simulink model "chbtask"  (R2024b)
settings: Solver=FixedStepDiscrete  StartTime=0.0  StopTime=0.2  FixedStep=5e-5  RelTol=1e-3
values from neighbouring files (symbols this model uses):
  CHB_MODE : value not decoded    [CHB_Data.sldd]
  INV120_CUURENTLOOP_KP = 2.0    [CHB_Data.sldd]
  INV120_CUURENTLOOP_KR = 5.0    [CHB_Data.sldd]
  INV120_VOLTAGELOOP_KI = 0.005    [CHB_Data.sldd]
  INV120_VOLTAGELOOP_KP = 0.5    [CHB_Data.sldd]
  INV240_VOLTAGELOOP_KI = 0.005    [CHB_Data.sldd]
  INV240_VOLTAGELOOP_KP = 0.5    [CHB_Data.sldd]
  PFC120_CUURENTLOOP_KP = 30.0    [CHB_Data.sldd]
  PFC120_CUURENTLOOP_KR = 8.0    [CHB_Data.sldd]
  PFC120_POWERLOOP_KI = 0.0001    [CHB_Data.sldd]
  PFC120_POWERLOOP_KP = 0.005    [CHB_Data.sldd]
  PFC240_CUURENTLOOP_KP = 5.0    [CHB_Data.sldd]
  PFC240_CUURENTLOOP_KR = 10.0    [CHB_Data.sldd]
  PFC240_POWERLOOP_KI = 0.0001    [CHB_Data.sldd]
  PFC240_POWERLOOP_KP = 0.005    [CHB_Data.sldd]
undefined symbols (not defined in the file or in its folder): Ii_rms, Io_rms, Io_rms_a, Io_rms_b, Vi_freq, Vi_rms, Vo_freq, Vo_freq_a, Vo_freq_b, Vo_rms, Vo_rms_a, Vo_rms_b
(part 2 of 3)

== system chbtask/Algorithm_Ctrl/MainCtrl/inv240_func/inv240_en ==
  note: 抗积分饱和
  note: 峰值限流保护是什么？？
  Bus Element In1 : Inport  PortName=Algorithm  Element=Vo_rms
  Enable : EnablePort
  Chart : Stateflow chart  TreatAsAtomicUnit=on
  Constant : Constant  Value=240  OutDataTypeStr=single
  Constant1 : Constant  Value=INV240_VOLTAGELOOP_KP  OutDataTypeStr=single
  Constant2 : Constant  Value=INV240_VOLTAGELOOP_KI  OutDataTypeStr=single
  Constant3 : Constant  Value=[360 100]  OutDataTypeStr=single
  Delay : Delay  DelayLength=1  InputProcessing=Columns as channels (frame based)
  Function Caller : FunctionCaller  FunctionPrototype=PI_out = Func.PI_Ctrl(error,err_sum,Kp,Ki,out_limit)  InputArgumentSpecifications=<Enter example>  OutputArgumentSpecifications=<Enter example>
  Mux : Mux  Inputs=2
  Saturation : Saturate  UpperLimit=360/INV240_VOLTAGELOOP_KI  LowerLimit=100/INV240_VOLTAGELOOP_KI
  Sum : Sum  Inputs=+-|
  Sum1 : Sum  Inputs=++|
  duty : Outport  OutDataTypeStr=single  PortDimensions=[1 2]
  wires:
  Constant/1 -> Sum/1
  Sum/1 -> Sum1/1, Function Caller/1
  Constant1/1 -> Function Caller/3
  Constant2/1 -> Function Caller/4
  Delay/1 -> Sum1/2
  Sum1/1 -> Saturation/1
  Constant3/1 -> Function Caller/5
  Function Caller/1 -> Chart/1(Pi_inv_out)
  Bus Element In1/1 -> Sum/2
  Mux/1 -> duty/1
  Chart/1(out) -> Mux/1, Mux/2
  Saturation/1 -> Delay/1, Function Caller/2

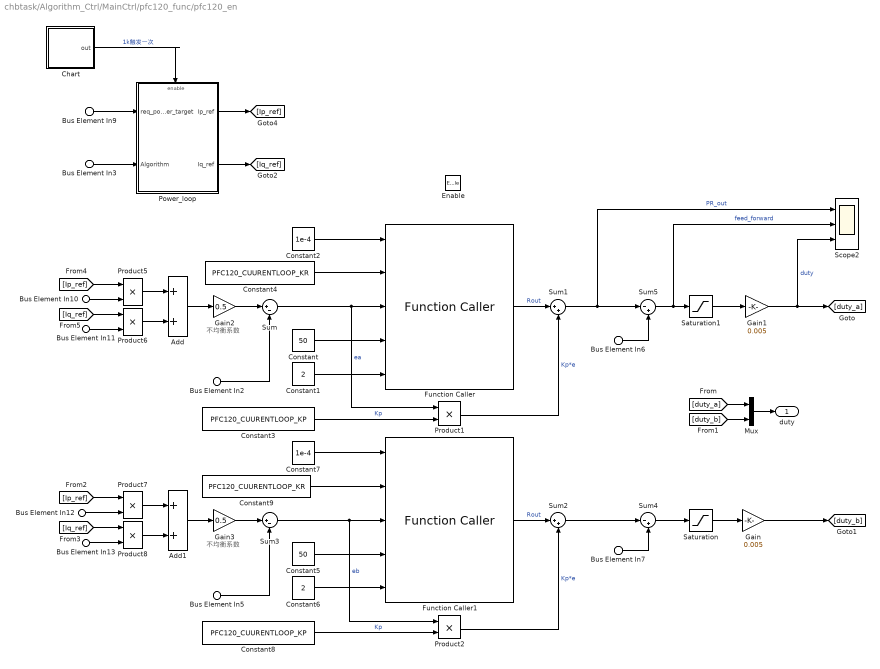
== system chbtask/Algorithm_Ctrl/MainCtrl/pfc120_func/pfc120_en ==
  note: 不均衡系数
  note: 不均衡系数
  Bus Element In10 : Inport  PortName=PLL  Element=cosin
  Bus Element In12 : Inport  PortName=PLL  Element=cosin
  Bus Element In11 : Inport  PortName=PLL  Element=sine
  Bus Element In13 : Inport  PortName=PLL  Element=sine
  Bus Element In2 : Inport  Port=2  PortName=Sampling  Element=AC_in_A.Igrid
  Bus Element In5 : Inport  Port=2  PortName=Sampling  Element=AC_in_B.Igrid
  Bus Element In6 : Inport  Port=2  PortName=Sampling  Element=AC_in.Vgrid
  Bus Element In7 : Inport  Port=2  PortName=Sampling  Element=AC_in.Vgrid
  Bus Element In9 : Inport  Port=2  PortName=Sampling  Element=AC_in.Power
  Bus Element In3 : Inport  Port=3  PortName=Algorithm
  Enable : EnablePort
  Add : Sum  OutDataTypeStr=single  AccumDataTypeStr=single
  Add1 : Sum  OutDataTypeStr=single  AccumDataTypeStr=single
  Chart : Stateflow chart  TreatAsAtomicUnit=on
  Constant : Constant  Value=50  OutDataTypeStr=single
  Constant1 : Constant  Value=2  OutDataTypeStr=single
  Constant2 : Constant  Value=1e-4  OutDataTypeStr=single
  Constant3 : Constant  Value=PFC120_CUURENTLOOP_KP  OutDataTypeStr=single
  Constant4 : Constant  Value=PFC120_CUURENTLOOP_KR  OutDataTypeStr=single
  Constant5 : Constant  Value=50  OutDataTypeStr=single
  Constant6 : Constant  Value=2  OutDataTypeStr=single
  Constant7 : Constant  Value=1e-4  OutDataTypeStr=single
  Constant8 : Constant  Value=PFC120_CUURENTLOOP_KP  OutDataTypeStr=single
  Constant9 : Constant  Value=PFC120_CUURENTLOOP_KR  OutDataTypeStr=single
  Function Caller : FunctionCaller  FunctionPrototype=R_out = Func.R_Ctrl(Ts,Kr,uk,freq0,freqc)  InputArgumentSpecifications=<Enter example>  OutputArgumentSpecifications=<Enter example>
  Function Caller1 : FunctionCaller  FunctionPrototype=R_out = Func.R_Ctrl(Ts,Kr,uk,freq0,freqc)  InputArgumentSpecifications=<Enter example>  OutputArgumentSpecifications=<Enter example>
  Gain : Gain  Gain=0.005  OutDataTypeStr=single
  Gain1 : Gain  Gain=0.005  OutDataTypeStr=single
  Gain2 : Gain  Gain=0.5  OutDataTypeStr=single
  Gain3 : Gain  Gain=0.5  OutDataTypeStr=single
  Mux : Mux  Inputs=2
  Power_loop : Subsystem
  Product1 : Product
  Product2 : Product
  Product{5..8} (4 alike) : Product  OutDataTypeStr=single
  Saturation : Saturate  UpperLimit=200  LowerLimit=-200  OutDataTypeStr=single
  Saturation1 : Saturate  UpperLimit=200  LowerLimit=-200  OutDataTypeStr=single
  Scope2 : Scope  NumInputPorts=3
  Sum : Sum  Inputs=|+-  OutDataTypeStr=single  AccumDataTypeStr=single
  Sum1 : Sum  Inputs=|++  OutDataTypeStr=single  AccumDataTypeStr=single
  Sum2 : Sum  Inputs=|++  OutDataTypeStr=single  AccumDataTypeStr=single
  Sum3 : Sum  Inputs=|+-
  Sum4 : Sum  Inputs=|-+  OutDataTypeStr=single  AccumDataTypeStr=single
  Sum5 : Sum  Inputs=|-+  OutDataTypeStr=single  AccumDataTypeStr=single
  duty : Outport  OutDataTypeStr=single  PortDimensions=[1 2]
  wires:
  Constant3/1 -> Product1/2  "Kp"
  Product1/1 -> Sum1/2  "Kp*e"
  Constant2/1 -> Function Caller/1
  Constant4/1 -> Function Caller/2
  Function Caller/1 -> Sum1/1  "Rout"
  Constant/1 -> Function Caller/4
  Constant1/1 -> Function Caller/5
  Constant6/1 -> Function Caller1/5
  Constant5/1 -> Function Caller1/4
  Function Caller1/1 -> Sum2/1  "Rout"
  Constant9/1 -> Function Caller1/2
  Constant7/1 -> Function Caller1/1
  Product2/1 -> Sum2/2  "Kp*e"
  Constant8/1 -> Product2/2  "Kp"
  Sum/1 -> Product1/1, Function Caller/3  "ea"
  Bus Element In2/1 -> Sum/2
  Sum3/1 -> Product2/1, Function Caller1/3  "eb"
  Bus Element In5/1 -> Sum3/2
  Mux/1 -> duty/1
  [duty_a] -> Mux/1
  [duty_b] -> Mux/2
  Sum2/1 -> Sum4/1
  Bus Element In7/1 -> Sum4/2
  Sum1/1 -> Scope2/1, Sum5/1  "PR_out"
  Bus Element In6/1 -> Sum5/2
  Saturation/1 -> Gain/1
  Sum4/1 -> Saturation/1
  Saturation1/1 -> Gain1/1
  Gain1/1 -> [duty_a], Scope2/3  "duty"
  Gain/1 -> [duty_b]
  Sum5/1 -> Scope2/2, Saturation1/1  "feed_forward"
  Chart/1(out) -> Power_loop/Enable  "1k触发一次"
  Bus Element In3/1 -> Power_loop/2(Algorithm)
  Bus Element In9/1 -> Power_loop/1(req_power_target)
  Bus Element In11/1 -> Product6/2
  Product6/1 -> Add/2
  Product5/1 -> Add/1
  [Iq_ref] -> Product6/1
  [Ip_ref] -> Product5/1
  Bus Element In10/1 -> Product5/2
  Power_loop/2(Iq_ref) -> [Iq_ref]
  Power_loop/1(Ip_ref) -> [Ip_ref]
  Add/1 -> Gain2/1
  Gain2/1 -> Sum/1
  Add1/1 -> Gain3/1
  Bus Element In12/1 -> Product7/2
  [Ip_ref] -> Product7/1
  [Iq_ref] -> Product8/1
  Product7/1 -> Add1/1
  Product8/1 -> Add1/2
  Bus Element In13/1 -> Product8/2
  Gain3/1 -> Sum3/1

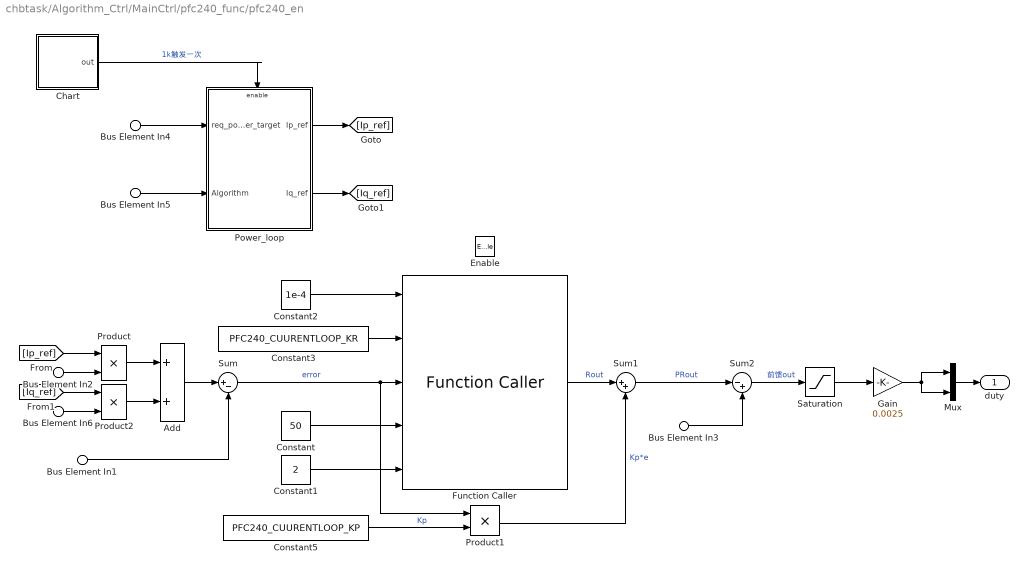
== system chbtask/Algorithm_Ctrl/MainCtrl/pfc240_func/pfc240_en ==
  Bus Element In2 : Inport  PortName=PLL  Element=cosin
  Bus Element In6 : Inport  PortName=PLL  Element=sine
  Bus Element In1 : Inport  Port=2  PortName=Sampling  Element=AC_in.Igrid
  Bus Element In3 : Inport  Port=2  PortName=Sampling  Element=AC_in.Vgrid
  Bus Element In4 : Inport  Port=2  PortName=Sampling  Element=AC_in.Power
  Bus Element In5 : Inport  Port=3  PortName=Algorithm
  Enable : EnablePort
  Add : Sum
  Chart : Stateflow chart  TreatAsAtomicUnit=on
  Constant : Constant  Value=50  OutDataTypeStr=single
  Constant1 : Constant  Value=2  OutDataTypeStr=single
  Constant2 : Constant  Value=1e-4  OutDataTypeStr=single
  Constant3 : Constant  Value=PFC240_CUURENTLOOP_KR  OutDataTypeStr=single
  Constant5 : Constant  Value=PFC240_CUURENTLOOP_KP  OutDataTypeStr=single
  Function Caller : FunctionCaller  FunctionPrototype=R_out = Func.R_Ctrl(Ts,Kr,uk,freq0,freqc)  InputArgumentSpecifications=<Enter example>  OutputArgumentSpecifications=<Enter example>
  Gain : Gain  Gain=0.0025  OutDataTypeStr=single
  Mux : Mux  Inputs=2
  Power_loop : Subsystem
  Product : Product  OutDataTypeStr=single
  Product1 : Product
  Product2 : Product  OutDataTypeStr=single
  Saturation : Saturate  UpperLimit=400  LowerLimit=-400  OutDataTypeStr=single
  Sum : Sum  Inputs=|+-  OutDataTypeStr=single  AccumDataTypeStr=single
  Sum1 : Sum  Inputs=|++  OutDataTypeStr=single  AccumDataTypeStr=single
  Sum2 : Sum  Inputs=|-+
  duty : Outport  OutDataTypeStr=single  PortDimensions=[1 2]
  wires:
  Constant1/1 -> Function Caller/5
  Constant/1 -> Function Caller/4
  Constant2/1 -> Function Caller/1
  Constant3/1 -> Function Caller/2
  Sum/1 -> Product1/1, Function Caller/3  "error"
  Bus Element In2/1 -> Product/2
  Constant5/1 -> Product1/2  "Kp"
  Function Caller/1 -> Sum1/1  "Rout"
  Product1/1 -> Sum1/2  "Kp*e"
  Saturation/1 -> Gain/1
  Sum1/1 -> Sum2/1  "PRout"
  Sum2/1 -> Saturation/1  "前馈out"
  Chart/1(out) -> Power_loop/Enable  "1k触发一次"
  Bus Element In1/1 -> Sum/2
  Bus Element In3/1 -> Sum2/2
  Bus Element In4/1 -> Power_loop/1(req_power_target)
  Bus Element In5/1 -> Power_loop/2(Algorithm)
  Power_loop/1(Ip_ref) -> [Ip_ref]
  [Ip_ref] -> Product/1
  Power_loop/2(Iq_ref) -> [Iq_ref]
  Bus Element In6/1 -> Product2/2
  Product2/1 -> Add/2
  Product/1 -> Add/1
  Add/1 -> Sum/1
  [Iq_ref] -> Product2/1
  Mux/1 -> duty/1
  Gain/1 -> Mux/2, Mux/1

== system chbtask/Algorithm_Ctrl/MainCtrl/inv120_func/inv120_en/Power_loop ==
  Vo_rms : Inport  OutDataTypeStr=single
  Enable : EnablePort
  Constant : Constant  Value=120  OutDataTypeStr=single
  Constant1 : Constant  Value=INV120_VOLTAGELOOP_KP  OutDataTypeStr=single
  Constant2 : Constant  Value=INV120_VOLTAGELOOP_KI  OutDataTypeStr=single
  Constant3 : Constant  Value=[30 0]  OutDataTypeStr=single
  Delay : Delay  DelayLength=1  InputProcessing=Columns as channels (frame based)
  Function Caller : FunctionCaller  FunctionPrototype=PI_out = Func.PI_Ctrl(error,err_sum,Kp,Ki,out_limit)  InputArgumentSpecifications=<Enter example>  OutputArgumentSpecifications=<Enter example>
  Scope : Scope
  Sum : Sum  Inputs=+-|
  Sum1 : Sum  Inputs=++|
  itotal_rms : Outport
  wires:
  Vo_rms/1 -> Sum/2
  Delay/1 -> Sum1/2
  Constant/1 -> Sum/1
  Constant3/1 -> Function Caller/5
  Sum1/1 -> Delay/1, Function Caller/2
  Sum/1 -> Sum1/1, Function Caller/1
  Function Caller/1 -> itotal_rms/1, Scope/1
  Constant2/1 -> Function Caller/4
  Constant1/1 -> Function Caller/3

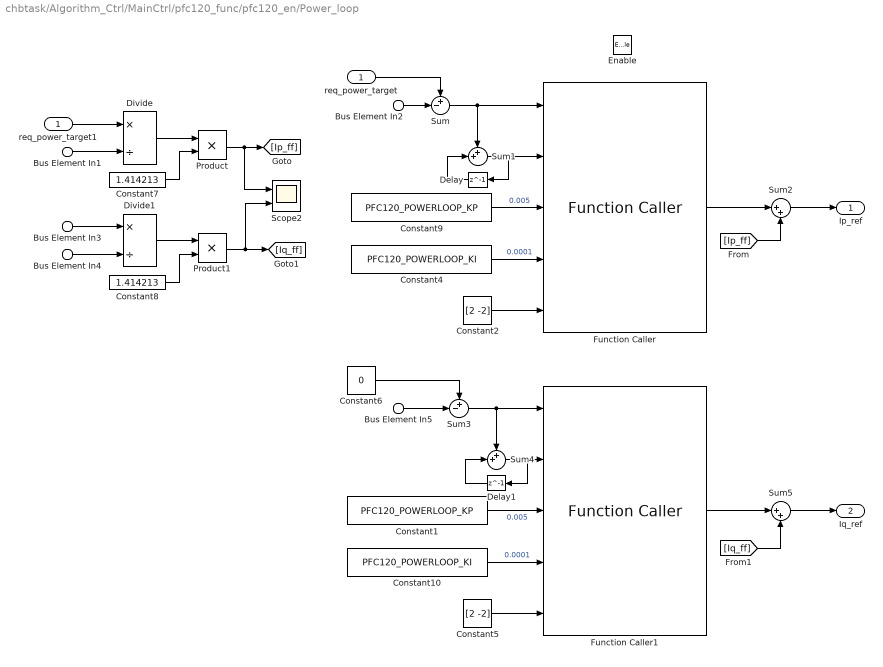
== system chbtask/Algorithm_Ctrl/MainCtrl/pfc120_func/pfc120_en/Power_loop ==
  req_power_target : Inport
  Bus Element In2 : Inport  Port=2  PortName=Algorithm  Element=pfc.P
  Bus Element In3 : Inport  Port=2  PortName=Algorithm  Element=pfc.Q
  Bus Element In5 : Inport  Port=2  PortName=Algorithm  Element=pfc.Q
  Bus Element In1 : Inport  Port=2  PortName=Algorithm  Element=Vi_rms
  Bus Element In4 : Inport  Port=2  PortName=Algorithm  Element=Vi_rms
  Enable : EnablePort
  Constant1 : Constant  Value=PFC120_POWERLOOP_KP  OutDataTypeStr=single
  Constant10 : Constant  Value=PFC120_POWERLOOP_KI  OutDataTypeStr=single
  Constant2 : Constant  Value=[2 -2]  OutDataTypeStr=single
  Constant4 : Constant  Value=PFC120_POWERLOOP_KI  OutDataTypeStr=single
  Constant5 : Constant  Value=[2 -2]  OutDataTypeStr=single
  Constant6 : Constant  Value=0  OutDataTypeStr=single
  Constant7 : Constant  Value=1.414213  OutDataTypeStr=single
  Constant8 : Constant  Value=1.414213  OutDataTypeStr=single
  Constant9 : Constant  Value=PFC120_POWERLOOP_KP  OutDataTypeStr=single
  Delay : Delay  DelayLength=1  InputProcessing=Columns as channels (frame based)
  Delay1 : Delay  DelayLength=1  InputProcessing=Columns as channels (frame based)
  Divide : Product  Inputs=*/  OutDataTypeStr=single
  Divide1 : Product  Inputs=*/  OutDataTypeStr=single
  Function Caller : FunctionCaller  FunctionPrototype=PI_out = Func.PI_Ctrl(error,err_sum,Kp,Ki,out_limit)  InputArgumentSpecifications=<Enter example>  OutputArgumentSpecifications=<Enter example>
  Function Caller1 : FunctionCaller  FunctionPrototype=PI_out = Func.PI_Ctrl(error,err_sum,Kp,Ki,out_limit)  InputArgumentSpecifications=<Enter example>  OutputArgumentSpecifications=<Enter example>
  Product : Product  OutDataTypeStr=single
  Product1 : Product  OutDataTypeStr=single
  Scope2 : Scope  NumInputPorts=2
  Sum : Sum  Inputs=+-|  OutDataTypeStr=single
  Sum1 : Sum  Inputs=++|  OutDataTypeStr=single
  Sum2 : Sum  Inputs=|++
  Sum3 : Sum  Inputs=+-|  OutDataTypeStr=single
  Sum4 : Sum  Inputs=++|  OutDataTypeStr=single
  Sum5 : Sum  Inputs=|++
  req_power_target1 : InportShadow
  Ip_ref : Outport
  Iq_ref : Outport  Port=2
  wires:
  Bus Element In2/1 -> Sum/2
  req_power_target/1 -> Sum/1
  Sum/1 -> Sum1/1, Function Caller/1
  Sum1/1 -> Delay/1, Function Caller/2
  Delay/1 -> Sum1/2
  Constant9/1 -> Function Caller/3  "0.005"
  Constant4/1 -> Function Caller/4  "0.0001"
  Constant2/1 -> Function Caller/5
  req_power_target1/1 -> Divide/1
  Bus Element In1/1 -> Divide/2
  Constant5/1 -> Function Caller1/5
  Delay1/1 -> Sum4/2
  Sum4/1 -> Function Caller1/2, Delay1/1
  Sum3/1 -> Function Caller1/1, Sum4/1
  Constant6/1 -> Sum3/1
  Bus Element In5/1 -> Sum3/2
  Bus Element In3/1 -> Divide1/1
  Bus Element In4/1 -> Divide1/2
  Function Caller1/1 -> Sum5/1
  [Iq_ff] -> Sum5/2
  Sum2/1 -> Ip_ref/1
  Function Caller/1 -> Sum2/1
  [Ip_ff] -> Sum2/2
  Divide/1 -> Product/1
  Constant7/1 -> Product/2
  Product/1 -> Scope2/1, [Ip_ff]
  Constant8/1 -> Product1/2
  Divide1/1 -> Product1/1
  Product1/1 -> Scope2/2, [Iq_ff]
  Sum5/1 -> Iq_ref/1
  Constant10/1 -> Function Caller1/4  "0.0001"
  Constant1/1 -> Function Caller1/3  "0.005"

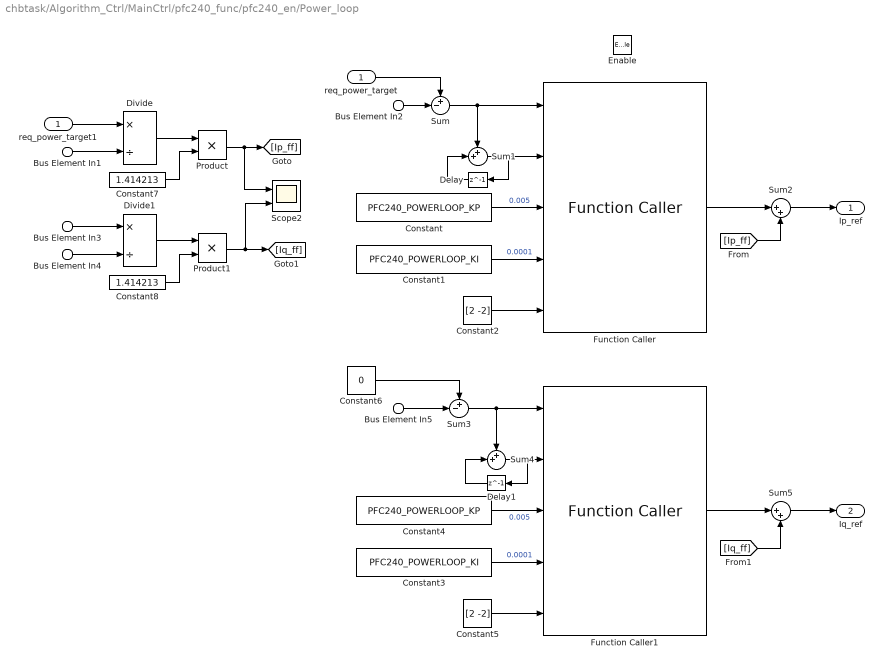
== system chbtask/Algorithm_Ctrl/MainCtrl/pfc240_func/pfc240_en/Power_loop ==
  req_power_target : Inport
  Bus Element In2 : Inport  Port=2  PortName=Algorithm  Element=pfc.P
  Bus Element In3 : Inport  Port=2  PortName=Algorithm  Element=pfc.Q
  Bus Element In5 : Inport  Port=2  PortName=Algorithm  Element=pfc.Q
  Bus Element In1 : Inport  Port=2  PortName=Algorithm  Element=Vi_rms
  Bus Element In4 : Inport  Port=2  PortName=Algorithm  Element=Vi_rms
  Enable : EnablePort
  Constant : Constant  Value=PFC240_POWERLOOP_KP  OutDataTypeStr=single
  Constant1 : Constant  Value=PFC240_POWERLOOP_KI  OutDataTypeStr=single
  Constant2 : Constant  Value=[2 -2]  OutDataTypeStr=single
  Constant3 : Constant  Value=PFC240_POWERLOOP_KI  OutDataTypeStr=single
  Constant4 : Constant  Value=PFC240_POWERLOOP_KP  OutDataTypeStr=single
  Constant5 : Constant  Value=[2 -2]  OutDataTypeStr=single
  Constant6 : Constant  Value=0  OutDataTypeStr=single
  Constant7 : Constant  Value=1.414213  OutDataTypeStr=single
  Constant8 : Constant  Value=1.414213  OutDataTypeStr=single
  Delay : Delay  DelayLength=1  InputProcessing=Columns as channels (frame based)
  Delay1 : Delay  DelayLength=1  InputProcessing=Columns as channels (frame based)
  Divide : Product  Inputs=*/  OutDataTypeStr=single
  Divide1 : Product  Inputs=*/  OutDataTypeStr=single
  Function Caller : FunctionCaller  FunctionPrototype=PI_out = Func.PI_Ctrl(error,err_sum,Kp,Ki,out_limit)  InputArgumentSpecifications=<Enter example>  OutputArgumentSpecifications=<Enter example>
  Function Caller1 : FunctionCaller  FunctionPrototype=PI_out = Func.PI_Ctrl(error,err_sum,Kp,Ki,out_limit)  InputArgumentSpecifications=<Enter example>  OutputArgumentSpecifications=<Enter example>
  Product : Product  OutDataTypeStr=single
  Product1 : Product  OutDataTypeStr=single
  Scope2 : Scope  NumInputPorts=2
  Sum : Sum  Inputs=+-|  OutDataTypeStr=single
  Sum1 : Sum  Inputs=++|  OutDataTypeStr=single
  Sum2 : Sum  Inputs=|++
  Sum3 : Sum  Inputs=+-|  OutDataTypeStr=single
  Sum4 : Sum  Inputs=++|  OutDataTypeStr=single
  Sum5 : Sum  Inputs=|++
  req_power_target1 : InportShadow
  Ip_ref : Outport
  Iq_ref : Outport  Port=2
  wires:
  Bus Element In2/1 -> Sum/2
  req_power_target/1 -> Sum/1
  Sum/1 -> Sum1/1, Function Caller/1
  Sum1/1 -> Delay/1, Function Caller/2
  Delay/1 -> Sum1/2
  Constant/1 -> Function Caller/3  "0.005"
  Constant1/1 -> Function Caller/4  "0.0001"
  Constant2/1 -> Function Caller/5
  req_power_target1/1 -> Divide/1
  Bus Element In1/1 -> Divide/2
  Constant5/1 -> Function Caller1/5
  Delay1/1 -> Sum4/2
  Sum4/1 -> Function Caller1/2, Delay1/1
  Sum3/1 -> Function Caller1/1, Sum4/1
  Constant6/1 -> Sum3/1
  Bus Element In5/1 -> Sum3/2
  Bus Element In3/1 -> Divide1/1
  Bus Element In4/1 -> Divide1/2
  Function Caller1/1 -> Sum5/1
  [Iq_ff] -> Sum5/2
  Sum2/1 -> Ip_ref/1
  Function Caller/1 -> Sum2/1
  [Ip_ff] -> Sum2/2
  Divide/1 -> Product/1
  Constant7/1 -> Product/2
  Product/1 -> Scope2/1, [Ip_ff]
  Constant8/1 -> Product1/2
  Divide1/1 -> Product1/1
  Product1/1 -> Scope2/2, [Iq_ff]
  Sum5/1 -> Iq_ref/1
  Constant3/1 -> Function Caller1/4  "0.0001"
  Constant4/1 -> Function Caller1/3  "0.005"

== stateflow chart chbtask/Algorithm_Ctrl/Data treating/SOGI/SOGI_Core ==
  state Run
    du:
    omega = 2*pi*single(50);
    T = single(1e-4);
    k = single(sqrt(2));
    e = vac - alpha_1 - k*beta_1;
    v_alpha = alpha_1 + T*omega*e;
    v_beta  = beta_1 + T*omega*v_alpha;
    alpha_1 = v_alpha;
    beta_1  = v_beta;
  (default) -> Run
  data: alpha_1 local single =0; beta_1 local single =0; omega local single =single(2*pi*50); T local single =single(1e-4); k local single =single(sqrt(2)); e local single; vac input single; v_alpha output single; v_beta output single

== stateflow chart chbtask/Algorithm_Ctrl/MainCtrl/pfc240_func/pfc240_en/Chart ==
  (default) -> (junction 8)
  (junction 8) -> (junction 6) [order 1] : [cnt>=9]
  (junction 8) -> (junction 10) [order 2] : {
      | out=0;
      | cnt = cnt + 1;
      | }
  (junction 6) -> (junction 11) : {
      | out=1;
      | cnt = 0;
      | }
  (junction 10) -> (junction 11)
  (junction 11) -> (junction 23)
  data: cnt local uint16 =0; out output uint16

== stateflow chart chbtask/Algorithm_Ctrl/MainCtrl/inv240_func/inv240_en/Chart ==
  (default) -> (junction 3) : {
      | pi_out_value = single(0.0025)*Pi_inv_out;
      | cnt = mod(cnt + 1, 200);
      | %PWM1 = sin_tab(mod(cnt + 0, 400) + 1);
      | out = pi_out_value*sin_wave(mod(cnt + 0, 200) + 1);
      | }
  data: sin_wave local single =[
0.000000000, 0.031410759, 0.062790520, 0.094108313, 0.125333234, 0.156434465, 0.187381315, 0.218143241, 0.248689887, 0.278991106, 0.309016994, 0.338737920, 0.368124553, 0.397147891, 0.425779292, 0.453990500, 0.481753674, 0.509041416, 0.535826795, 0.562083325, 0.587785252, 0.612907054, 0.637423990, 0.661311865, 0.684547106, 0.707106781, 0.728968627, 0.750111065, 0.770513243, 0.790155012, 0.809016994, 0.827080574, 0.844327926, 0.860742028, 0.876306680, 0.891006524, 0.904827052, 0.917754626, 0.929776486, 0.940880769, 0.951056516, 0.960293686, 0.968583162, 0.975916762, 0.982287251, 0.987688341, 0.992114701, 0.995561965, 0.998026728, 0.999506560, 1.000000000, 0.999506560, 0.998026728, 0.995561965, 0.992114701, 0.987688341, 0.982287251, 0.975916762, 0.968583162, 0.960293686, 0.951056516, 0.940880769, 0.929776486, 0.917754626, 0.904827052, 0.891006524, 0.876306680, 0.860742028, 0.844327926, 0.827080574, 0.809016994, 0.790155012, 0.770513243, 0.750111065, 0.728968627, 0.707106781, 0.684547106, 0.661311865, 0.637423990, 0.612907054, 0.587785252, 0.562083325, 0.535826795, 0.509041416, 0.481753674, 0.453990500, 0.425779292, 0.397147891, 0.368124553, 0.338737920, 0.309016994, 0.278991106, 0.248689887, 0.218143241, 0.187381315, 0.156434465, 0.125333234, 0.094108313, 0.062790520, 0.031410759, 0.000000000, -0.031410759, -0.062790520, -0.094108313, -0.125333234, -0.156434465, -0.187381315, -0.218143241, -0.248689887, -0.278991106, -0.309016994, -0.338737920, -0.368124553, -0.397147891, -0.425779292, -0.453990500, -0.481753674, -0.509041416, -0.535826795, -0.562083325, -0.587785252, -0.612907054, -0.637423990, -0.661311865, -0.684547106, -0.707106781, -0.728968627, -0.750111065, -0.770513243, -0.790155012, -0.809016994, -0.827080574, -0.844327926, -0.860742028, -0.876306680, -0.891006524, -0.904827052, -0.917754626, -0.929776486, -0.940880769, -0.951056516, -0.960293686, -0.968583162, -0.975916762, -0.982287251, -0.987688341, -0.992114701, -0.995561965, -0.998026728, -0.999506560, -1.000000000, -0.999506560, -0.998026728, -0.995561965, -0.992114701, -0.987688341, -0.982287251, -0.975916762, -0.968583162, -0.960293686, -0.951056516, -0.940880769, -0.929776486, -0.917754626, -0.904827052, -0.891006524, -0.876306680, -0.860742028, -0.844327926, -0.827080574, -0.809016994, -0.790155012, -0.770513243, -0.750111065, -0.728968627, -0.707106781, -0.684547106, -0.661311865, -0.637423990, -0.612907054, -0.587785252, -0.562083325, -0.535826795, -0.509041416, -0.481753674, -0.453990500, -0.425779292, -0.397147891, -0.368124553, -0.338737920, -0.309016994, -0.278991106, -0.248689887, -0.218143241, -0.187381315, -0.156434465, -0.125333234, -0.094108313, -0.062790520, -0.031410759
]; Pi_inv_out input single; cnt local single =0; out output single =0; pi_out_value local single =0

== stateflow chart chbtask/Algorithm_Ctrl/MainCtrl/pfc240_func/Chart ==
  state init_state
    en:
    cnt = uint16(0);
    run_en = false;
  state en_run
    du:
    cnt = cnt+uint16(1);
    if cnt>=500
    run_en = true;
    cnt = uint16(500);
    else
    run_en = false;
    end
  (default) -> init_state
  init_state -> en_run : [En_PFC240==1]
  en_run -> init_state : [En_PFC240==0]
  data: cnt local uint16 =0; En_PFC240 input; run_en output boolean

== stateflow chart chbtask/Algorithm_Ctrl/MainCtrl/Subsystem/Chart ==
  state Standby
    du:
    Relay.jk1 = false;
    Relay.jk2 = false;
    Relay.jk3 = false;
    Relay.jk4 = false;
    Relay.jk5 = false;
    Relay.jk6 = false;
    Relay.jk7 = false;
    Relay.jk8 = false;
    Relay.jk9 = false;
  state Pfc120
    Relay.jk1 = true;
    Relay.jk2 = true;
    Relay.jk3 = false;
    Relay.jk4 = true;
    Relay.jk5 = false;
    Relay.jk6 = false;
    Relay.jk7 = false;
    Relay.jk8 = false;
    Relay.jk9 = false;
  state Pfc240
    Relay.jk1 = false;
    Relay.jk2 = false;
    Relay.jk3 = true;
    Relay.jk4 = true;
    Relay.jk5 = false;
    Relay.jk6 = false;
    Relay.jk7 = false;
    Relay.jk8 = false;
    Relay.jk9 = false;
  state Inv240
    Relay.jk1 = false;
    Relay.jk2 = false;
    Relay.jk3 = true;
    Relay.jk4 = false;
    Relay.jk5 = true;
    Relay.jk6 = false;
    Relay.jk7 = true;
    Relay.jk8 = true;
    Relay.jk9 = true;
  state Inv120
    Relay.jk1 = false;
    Relay.jk2 = false;
    Relay.jk3 = false;
    Relay.jk4 = false;
    Relay.jk5 = false;
    Relay.jk6 = true;
    Relay.jk7 = false;
    Relay.jk8 = true;
    Relay.jk9 = true;
  (default) -> Standby
  Standby -> Pfc120 [order 4] : [CMD_Model == CHB_MODE.PFC120 && stabflg==true]
  Pfc120 -> Standby : [CMD_Model == CHB_MODE.STANDBY || stabflg==false]
  Pfc240 -> Standby : [CMD_Model == CHB_MODE.STANDBY || stabflg==false]
  Standby -> Pfc240 [order 3] : [CMD_Model == CHB_MODE.PFC240 && stabflg==true]
  Standby -> Inv240 [order 1] : [CMD_Model == CHB_MODE.INV240 && stabflg==true]
  Inv240 -> Standby : [CMD_Model == CHB_MODE.STANDBY || stabflg==false]
  Inv120 -> Standby : [CMD_Model == CHB_MODE.STANDBY || stabflg==false]
  Standby -> Inv120 [order 2] : [CMD_Model == CHB_MODE.INV120 && stabflg==true]
  data: stabflg input; CMD_Model input Enum: CHB_MODE; Relay output Bus: Relay_t

== stateflow chart chbtask/Func/Simulink Function9/Chart ==
  (default) -> (junction 4) : {
      | out = factor*input +(single(1) - factor)*out_pre;
      | %out_pre = out;
      | }
  data: input input single; factor input single; out output single; out_pre input single =0

== stateflow chart chbtask/Func/Simulink Function/Chart ==
  state sogi_init
    omiga = 2*pi*wt;
    cons_x=2*k*omiga*T;
    cons_y=omiga*omiga*T*T;
    cons_z=1/(cons_x+cons_y+4);
    a1=2*(4-cons_y)*cons_z;
    a2=(cons_x-cons_y-4)*cons_z;
    b0=cons_x*cons_z;
    bq=k*cons_y*cons_z;
    ex:
    wt1=wt;
  state sogi_run
    du:
    alpha=(b0*uk)-(b0*uk_2)+(a1*alpha_1)+(a2*alpha_2);
    beta=(bq*uk)+(2*bq*uk_1)+(bq*uk_2)+(a1*beta_1)+(a2*beta_2);
    uk_2=uk_1;
    uk_1=uk;
    alpha_2=alpha_1;
    alpha_1=alpha;
    beta_2=beta_1;
    beta_1=beta;
  (default) -> sogi_init
  sogi_init -> sogi_run
  sogi_run -> sogi_init : [wt~=wt1]
  data: uk input single; wt input single; k input single; T input single; alpha output single =0; beta output single =0; omiga local single =0; cons_x local single =0; cons_y local single =0; a1 local single =0; a2 local single =0; b0 local single =0; bq local single =0; wt1 local single =0; alpha_2 local single =0; beta_2 local single =0; alpha_1 local single =0; beta_1 local single =0; uk_1 local single =0; uk_2 local single =0; cons_z local single =0

== matlab function chbtask/Func/Simulink Function1/MATLAB Function ==
  data: fault_in input boolean; recover_in input boolean; fault_cnt input int16; recover_cnt input int16; lock_en input boolean; fault_en input uint32; cnt input int16; fault_en output; cnt output
function [fault_en,cnt]= fault_detect(fault_in, recover_in, fault_cnt, recover_cnt, lock_en, fault_en, cnt)
if lock_en && (fault_en==uint32(1))
    fault_en=uint32(1);
    return;
end
%%考虑边界防抖动
if fault_in 
    cnt = cnt + int16(1);    
elseif ~fault_in
    cnt = cnt-int16(1);
end
if cnt >= fault_cnt
   fault_en=uint32(1);
   cnt=int16(0);
end

if recover_in 
   cnt = cnt-int16(1);
elseif ~recover_in
cnt = cnt + int16(1);
end
if cnt <= (-recover_cnt)
fault_en=uint32(0);
cnt=int16(0);
end
cnt=max(cnt, fault_cnt);
cnt=min(cnt, -recover_cnt);

== stateflow chart chbtask/Func/Simulink Function2/Chart ==
  state sogi_init
    omiga=wt*2*pi;
    cons_a=omiga*omiga*T*T;
    cons_b = k*omiga*T;
    cons_c=k*cons_a;
    cons_d=1/(1+cons_b+cons_a);
    a1=single(-1)*(2+cons_b)*cons_d;
    a2=single(1)*cons_d;
    b0=cons_b*cons_d;
    bq=cons_c*cons_d;
    ex:
    wtk_1=wt;
  state sogi_run
    du:
    alpha=(b0*uk)-(b0*uk_1)-(a1*alpha_1)-(a2*alpha_2);
    beta=(bq*uk)-(a1*beta_1)-(a2*beta_2);
    uk_1=uk;
    alpha_2=alpha_1;
    beta_2=beta_1;
    alpha_1=alpha;
    beta_1=beta;
  (default) -> sogi_init
  sogi_init -> sogi_run
  sogi_run -> sogi_init : [wt~=wtk_1]
  data: uk input single; wt input single; k input single; T input single; cons_b local single =0; cons_a local single =0; omiga local single =0; cons_c local single =0; cons_d local single =0; a1 local single =0; a2 local single =0; b0 local single =0; bq local single =0; uk_1 local single =0; alpha output single =0; beta output single =0; alpha_1 local single =0; alpha_2 local single =0; beta_1 local single =0; beta_2 local single =0; wtk_1 local single =0

== stateflow chart chbtask/Func/Simulink Function3/Chart ==
  note: k直接取1后的表达式：
      | $Y_\alpha(k) = Y_\alpha(k-1)+T\omega_o e(k-1)$
      | $Y_\beta(k) = Y_\beta(k-1) + T\omega_0 Y_\alpha(k-1)$
      | $e(k) = u(k)-Y_\alpha(k)-Y_\beta(k)$
      | 这里需要注意一下，尽管公式推导用的是alpha(k-1),
      | 但是beta本质上是由当前的alpha输出影响的，
      | 而非上一时刻的alpha，系统能不滞后就不要滞后，时效性要好。
      | 仿真也确实带了两个alpha进去，当前alpha的效果确实更好
      | 所以最终的输出公式为：
      | $Y_\alpha(k) = Y_\alpha(k-1)+T\omega_o e(k-1)$
      | $Y_\beta(k) = Y_\beta(k-1) + T\omega_0 Y_\alpha(k )$
      | $e(k) = u(k)-Y_\alpha(k)-Y_\beta(k)$
  (default) -> (junction 16) : {
      | omega = 2*pi*wt;
      | e=uk-alpha_1-beta_1;
      | alpha = alpha_1 + T*omega*e;
      | beta = beta_1+T*omega*alpha;
      | }
  data: alpha output; beta output; uk input; wt input single; T input; omega local single =0; e local single =0; alpha_1 input single =0; beta_1 input single =0

== stateflow chart chbtask/Func/Simulink Function5/Chart ==
  (default) -> (junction 17) : {
      | %y(k) = p*e(k) + i *∑ e(k)
      | %e(k) = 目标值(k)-实际值(k)
      |
      | %e_sum = e_sum + error;
      | I_out = e_sum * Ki;
      | P_out = error*Kp;
      | out_0 = P_out + I_out;
      | }
  (junction 17) -> (junction 21) [order 1] : [out_0>limit(1)]
  (junction 21) -> (junction 27) : {out = limit(1)}
  (junction 17) -> (junction 23) [order 2] : [out_0<limit(2)]
  (junction 17) -> (junction 25) [order 3] : {out = out_0;}
  (junction 27) -> (junction 28)
  (junction 23) -> (junction 28) : {out = limit(2)}
  (junction 28) -> (junction 25)
  (junction 25) -> (junction 31)
  data: error input single; e_sum input single; Kp input single; Ki input single; out output single =0; limit input single size=[1 2]; I_out local single =0; P_out local single =0; out_0 local single =0

== stateflow chart chbtask/Func/Simulink Function7/R ==
  state Init
    en:
    omiga0 = 2*pi*freq0;
    omigac = 2*pi*freqc;
    x = omigac*Ts;
    y = omiga0*omiga0*Ts*Ts;
    z = single(1)/(4 + 4 * x + y);
    b0 = 4 * Kr * x * z;
    b1 = single(-1) * b0;
    a0 = (2 * y - 8) * z;
    a1 = (4 - 4 * x + y) * z;
    ex:
    pre_freq0 = freq0;
    pre_freqc = freqc;
  state R_Ctrl
    du:
    yk = b0*uk + b1*uk_2 - a0*yk_1 - a1*yk_2;
    uk_2 = uk_1;
    uk_1 = uk;
    yk_2 = yk_1;
    yk_1 = yk;
  (default) -> Init
  Init -> R_Ctrl
  R_Ctrl -> Init : [freq0~=pre_freq0 || freqc~= pre_freqc]
  data: Ts input single; Kr input single; uk input single; freq0 input single; freqc input single; omiga0 local single; omigac local single; a0 local single; b0 local single; x local single; y local single; z local single; b1 local single; a1 local single; yk output single; yk_2 local single =0; yk_1 local single =0; uk_1 local single =0; pre_freqc local single; pre_freq0 local single; uk_2 local single =0

== stateflow chart chbtask/Func/Simulink Function4/Chart1 ==
  (default) -> (junction 17) : {
      | %y(k) = p*e(k) + i *∑ e(k)
      | %e(k) = 目标值(k)-实际值(k)
      | e_sum = e_sum + error;
      | I_out = e_sum * Ki;
      | P_out = error*Kp;
      | out = P_out + I_out;
      | }
  data: Kp input single; Ki input single; error input single; out output single =0; e_sum local single =0; I_out local single =0; P_out local single =0

== stateflow chart chbtask/Func/Simulink Function4/Chart ==
  note: 外面那个2e-4的增益，是基于另一个模型theta-mod步进得到的，发现pi_out第一个输出是≈2e-4,所以才有这个增益的，因为uk有个100pi累加，第一个输出>=100pi，当前系统周期为10k，这个要1.5个周期才能锁相，P取100，I取50，没有mod这种除法函数，uk、persun、theta都不会溢出
  (default) -> (junction 15) : {
      | pre_sum = pre_sum + uk;
      | }
  (junction 15) -> (junction 17) [order 1] : [pre_sum>single(2*pi)]
  (junction 15) -> (junction 21) [order 2]
  (junction 17) -> (junction 19) : {pre_sum = pre_sum-single(2*pi);}
  (junction 19) -> (junction 21)
  (junction 21) -> (junction 24) : {theta = pre_sum;}
  data: uk input single; theta output single =0; pre_sum local single =0

== stateflow chart chbtask/Func/Simulink Function4/Chart2 ==
  (default) -> (junction 8) : {
      | %有mod这种复杂的运算，看情况用吧，半个周期就能追上，
      | %当前系统周期10kHz,p=0.4, i=0.8
      | %uk、persun、theta都不会溢出
      | pre_sum = mod(pre_sum + uk, 2*pi);
      | theta = pre_sum;
      | }
  data: uk input single; theta output single =0; pre_sum local single =0

== stateflow chart chbtask/Func/Simulink Function6/Chart1 ==
  (default) -> (junction 1) : {Pk = Uk*Ik;}
  (junction 15) -> (junction 33) [order 2]
  (junction 9) -> (junction 15) [order 1] : [Uk-Uk_1>0]
      | {%正向爬坡
      | positive = positive+1;
      | }
  (junction 1) -> (junction 9) [order 2]
  (junction 1) -> (junction 6) [order 1] : [Pk<=Pk_1]
  (junction 6) -> (junction 12) [order 1] : [Uk-Uk_1>0]
      | {negative = negative+1;}
  (junction 12) -> (junction 38) [order 2]
  (junction 33) -> (junction 35) : {
      | Uref = Uref+Ustep;
      | }
  (junction 15) -> (junction 17) [order 1] : [positive>=3]
  (junction 9) -> (junction 18) [order 2] : {%反向爬坡接近山顶了，变小步长
      | positive = 0;}
  (junction 6) -> (junction 19) [order 2] : {%正向爬山接近山顶了,变小步长
      | negative = 0;}
  (junction 12) -> (junction 20) [order 1] : [negative>=3]
  (junction 38) -> (junction 42) : {
      | Uref = Uref - Ustep;
      | }
  (junction 17) -> (junction 30) : {
      | %连续三次获得正反馈可跨大步长
      | Uref = Uref+Ustep*single(1.2);
      | }
  (junction 18) -> (junction 27) : {Uref = Uref-Ustep*single(0.5);}
  (junction 19) -> (junction 25) : {Uref = Uref+Ustep*single(0.5);}
  (junction 20) -> (junction 40) : {%连续三次获得负反馈可跨大步长
      | Uref = Uref-Ustep*single(1.2);
      | }
  (junction 35) -> (junction 30)
  (junction 30) -> (junction 27)
  (junction 27) -> (junction 44)
  (junction 25) -> (junction 44)
  (junction 40) -> (junction 25)
  (junction 42) -> (junction 40)
  (junction 44) -> (junction 51) : {Uk_1=Uk;
      | Pk_1 = Pk;}
  data: Uk input single; Ik input single; Ustep input single; Pk_1 local single =0; Pk local single =0; Uk_1 local single =0; positive local single =0; Uref output single =0; negative local single =0

== stateflow chart chbtask/Algorithm_Ctrl/MainCtrl/inv120_func/inv120_en/Chart ==
  (default) -> (junction 3) : {
      | pi_out_value = single(1)*Pi_inv_out;
      | cnt = mod(cnt + 1, 200);
      | %PWM1 = sin_tab(mod(cnt + 0, 400) + 1);
      | out = pi_out_value*sin_wave(mod(cnt + 0, 200) + 1);
      | }
  data: sin_wave local single =[
0.000000000, 0.031410759, 0.062790520, 0.094108313, 0.125333234, 0.156434465, 0.187381315, 0.218143241, 0.248689887, 0.278991106, 0.309016994, 0.338737920, 0.368124553, 0.397147891, 0.425779292, 0.453990500, 0.481753674, 0.509041416, 0.535826795, 0.562083325, 0.587785252, 0.612907054, 0.637423990, 0.661311865, 0.684547106, 0.707106781, 0.728968627, 0.750111065, 0.770513243, 0.790155012, 0.809016994, 0.827080574, 0.844327926, 0.860742028, 0.876306680, 0.891006524, 0.904827052, 0.917754626, 0.929776486, 0.940880769, 0.951056516, 0.960293686, 0.968583162, 0.975916762, 0.982287251, 0.987688341, 0.992114701, 0.995561965, 0.998026728, 0.999506560, 1.000000000, 0.999506560, 0.998026728, 0.995561965, 0.992114701, 0.987688341, 0.982287251, 0.975916762, 0.968583162, 0.960293686, 0.951056516, 0.940880769, 0.929776486, 0.917754626, 0.904827052, 0.891006524, 0.876306680, 0.860742028, 0.844327926, 0.827080574, 0.809016994, 0.790155012, 0.770513243, 0.750111065, 0.728968627, 0.707106781, 0.684547106, 0.661311865, 0.637423990, 0.612907054, 0.587785252, 0.562083325, 0.535826795, 0.509041416, 0.481753674, 0.453990500, 0.425779292, 0.397147891, 0.368124553, 0.338737920, 0.309016994, 0.278991106, 0.248689887, 0.218143241, 0.187381315, 0.156434465, 0.125333234, 0.094108313, 0.062790520, 0.031410759, 0.000000000, -0.031410759, -0.062790520, -0.094108313, -0.125333234, -0.156434465, -0.187381315, -0.218143241, -0.248689887, -0.278991106, -0.309016994, -0.338737920, -0.368124553, -0.397147891, -0.425779292, -0.453990500, -0.481753674, -0.509041416, -0.535826795, -0.562083325, -0.587785252, -0.612907054, -0.637423990, -0.661311865, -0.684547106, -0.707106781, -0.728968627, -0.750111065, -0.770513243, -0.790155012, -0.809016994, -0.827080574, -0.844327926, -0.860742028, -0.876306680, -0.891006524, -0.904827052, -0.917754626, -0.929776486, -0.940880769, -0.951056516, -0.960293686, -0.968583162, -0.975916762, -0.982287251, -0.987688341, -0.992114701, -0.995561965, -0.998026728, -0.999506560, -1.000000000, -0.999506560, -0.998026728, -0.995561965, -0.992114701, -0.987688341, -0.982287251, -0.975916762, -0.968583162, -0.960293686, -0.951056516, -0.940880769, -0.929776486, -0.917754626, -0.904827052, -0.891006524, -0.876306680, -0.860742028, -0.844327926, -0.827080574, -0.809016994, -0.790155012, -0.770513243, -0.750111065, -0.728968627, -0.707106781, -0.684547106, -0.661311865, -0.637423990, -0.612907054, -0.587785252, -0.562083325, -0.535826795, -0.509041416, -0.481753674, -0.453990500, -0.425779292, -0.397147891, -0.368124553, -0.338737920, -0.309016994, -0.278991106, -0.248689887, -0.218143241, -0.187381315, -0.156434465, -0.125333234, -0.094108313, -0.062790520, -0.031410759
]; Pi_inv_out input single; cnt local single =0; out output single =0; pi_out_value local single =0

== stateflow chart chbtask/Func/Simulink Function10/Chart ==
  note: 无功功率: $q=\frac{1}{2}(u_{\alpha}i_{\beta}-u_{\beta}i_{\alpha})$ q有时候定义是反相的，根据需求决定
      | 有功功率: $p=\frac{1}{2}(u_{\alpha}i_{\alpha}+u_{\beta}i_{\beta})$
  (default) -> (junction 3) : {
      | q = single(0.5)*(beta(1)*alpha(2) - alpha(1)*beta(2));
      | p = single(0.5)*(alpha(1)*alpha(2)+beta(1)*beta(2));
      | }
  data: alpha input single size=[1 2]; beta input single size=[1 2]; q output single =0; p output single =0

== stateflow chart chbtask/Algorithm_Ctrl/MainCtrl/pfc120_func/Chart ==
  state init_state
    en:
    cnt = uint16(0);
    run_en = false;
  state en_run
    du:
    cnt = cnt+uint16(1);
    if cnt>=500
    run_en = true;
    cnt = uint16(500);
    else
    run_en = false;
    end
  (default) -> init_state
  init_state -> en_run : [En_PFC120==1]
  en_run -> init_state : [En_PFC120==0]
  data: cnt local uint16 =0; En_PFC120 input; run_en output boolean

== stateflow chart chbtask/Algorithm_Ctrl/MainCtrl/pfc120_func/pfc120_en/Chart ==
  (default) -> (junction 8)
  (junction 8) -> (junction 6) [order 1] : [cnt>=9]
  (junction 8) -> (junction 10) [order 2] : {
      | out=0;
      | cnt = cnt + 1;
      | }
  (junction 6) -> (junction 11) : {
      | out=1;
      | cnt = 0;
      | }
  (junction 10) -> (junction 11)
  (junction 11) -> (junction 23)
  data: cnt local uint16 =0; out output uint16

== stateflow chart chbtask/Algorithm_Ctrl/MainCtrl/inv120_func/inv120_en/Chart2 ==
  (default) -> (junction 8)
  (junction 8) -> (junction 6) [order 1] : [cnt>=9]
  (junction 8) -> (junction 10) [order 2] : {
      | out=0;
      | cnt = cnt + 1;
      | }
  (junction 6) -> (junction 11) : {
      | out=1;
      | cnt = 0;
      | }
  (junction 10) -> (junction 11)
  (junction 11) -> (junction 23)
  data: cnt local uint16 =0; out output uint16

== stateflow chart chbtask/Func/Simulink Function11/Chart ==
  (default) -> (junction 4)
  (junction 4) -> (junction 7) [order 2] : [input>limit(2)]
  (junction 7) -> (junction 11) : {out = limit(2);}
  (junction 4) -> (junction 18) [order 1] : [input<limit(1)]
  (junction 4) -> (junction 9) [order 3] : {out = input}
  (junction 11) -> (junction 17)
  (junction 18) -> (junction 17) : {out = limit(1);}
  (junction 17) -> (junction 9)
  (junction 9) -> (junction 14)
  data: input input single; limit input single size=[1 2]; out output single

== stateflow chart chbtask/Algorithm_Ctrl/MainCtrl/inv120_func/inv120_en/Chart6 ==
  (default) -> (junction 3) : {
      | pi_out_value = single(1)*Pi_inv_out;
      | cnt = mod(cnt + 1, 200);
      | %PWM1 = sin_tab(mod(cnt + 0, 400) + 1);
      | out = pi_out_value*sin_wave(mod(cnt + 0, 200) + 1);
      | }
  data: sin_wave local single =[
0.000000000, 0.031410759, 0.062790520, 0.094108313, 0.125333234, 0.156434465, 0.187381315, 0.218143241, 0.248689887, 0.278991106, 0.309016994, 0.338737920, 0.368124553, 0.397147891, 0.425779292, 0.453990500, 0.481753674, 0.509041416, 0.535826795, 0.562083325, 0.587785252, 0.612907054, 0.637423990, 0.661311865, 0.684547106, 0.707106781, 0.728968627, 0.750111065, 0.770513243, 0.790155012, 0.809016994, 0.827080574, 0.844327926, 0.860742028, 0.876306680, 0.891006524, 0.904827052, 0.917754626, 0.929776486, 0.940880769, 0.951056516, 0.960293686, 0.968583162, 0.975916762, 0.982287251, 0.987688341, 0.992114701, 0.995561965, 0.998026728, 0.999506560, 1.000000000, 0.999506560, 0.998026728, 0.995561965, 0.992114701, 0.987688341, 0.982287251, 0.975916762, 0.968583162, 0.960293686, 0.951056516, 0.940880769, 0.929776486, 0.917754626, 0.904827052, 0.891006524, 0.876306680, 0.860742028, 0.844327926, 0.827080574, 0.809016994, 0.790155012, 0.770513243, 0.750111065, 0.728968627, 0.707106781, 0.684547106, 0.661311865, 0.637423990, 0.612907054, 0.587785252, 0.562083325, 0.535826795, 0.509041416, 0.481753674, 0.453990500, 0.425779292, 0.397147891, 0.368124553, 0.338737920, 0.309016994, 0.278991106, 0.248689887, 0.218143241, 0.187381315, 0.156434465, 0.125333234, 0.094108313, 0.062790520, 0.031410759, 0.000000000, -0.031410759, -0.062790520, -0.094108313, -0.125333234, -0.156434465, -0.187381315, -0.218143241, -0.248689887, -0.278991106, -0.309016994, -0.338737920, -0.368124553, -0.397147891, -0.425779292, -0.453990500, -0.481753674, -0.509041416, -0.535826795, -0.562083325, -0.587785252, -0.612907054, -0.637423990, -0.661311865, -0.684547106, -0.707106781, -0.728968627, -0.750111065, -0.770513243, -0.790155012, -0.809016994, -0.827080574, -0.844327926, -0.860742028, -0.876306680, -0.891006524, -0.904827052, -0.917754626, -0.929776486, -0.940880769, -0.951056516, -0.960293686, -0.968583162, -0.975916762, -0.982287251, -0.987688341, -0.992114701, -0.995561965, -0.998026728, -0.999506560, -1.000000000, -0.999506560, -0.998026728, -0.995561965, -0.992114701, -0.987688341, -0.982287251, -0.975916762, -0.968583162, -0.960293686, -0.951056516, -0.940880769, -0.929776486, -0.917754626, -0.904827052, -0.891006524, -0.876306680, -0.860742028, -0.844327926, -0.827080574, -0.809016994, -0.790155012, -0.770513243, -0.750111065, -0.728968627, -0.707106781, -0.684547106, -0.661311865, -0.637423990, -0.612907054, -0.587785252, -0.562083325, -0.535826795, -0.509041416, -0.481753674, -0.453990500, -0.425779292, -0.397147891, -0.368124553, -0.338737920, -0.309016994, -0.278991106, -0.248689887, -0.218143241, -0.187381315, -0.156434465, -0.125333234, -0.094108313, -0.062790520, -0.031410759
]; Pi_inv_out input single; cnt local single =0; out output single =0; pi_out_value local single =0
